simulink model "Model_LQR_Real_First_order"  (R2025a)
settings: Solver=ode4  StartTime=0.0  StopTime=2  FixedStep=0.0001  RelTol=1e-3
InitFcn:
  | addpath('functions');
model workspace: external: MATLAB File D:\OneDrive - University of Bristol\2025-2026\Major Project\LQR\LQR_First_order\Discrete_of_init_LQR.m (data not in the file)
values from neighbouring files (symbols this model uses):
  alpha_angle = 0.9    [Discrete_of_init_LQR.m]
  alpha_output = 0.71    [Discrete_of_init_LQR.m]
  c_omega = (N_gear^2 * Kt * Ke) / R_motor    (= 0.00492477886361)    [Discrete_of_init_LQR.m]    (also in init_LQR.m)
  c_V = (N_gear * Kt) / R_motor    (= 0.0277237642805)    [Discrete_of_init_LQR.m]    (also in init_LQR.m)
  dist_duration = 0    [L_curve.m]
  fric_1 = [f_v_1, f_c_1, k_fc_1]    [Discrete_of_init_LQR.m]    (also in furuta_single_inverted_pendulum_nonlive_copy.m; init_LQR.m)
  fric_arm = [f_v_arm, f_c_arm, k_fc_arm]    [Discrete_of_init_LQR.m]    (also in furuta_single_inverted_pendulum_nonlive_copy.m; init_LQR.m)
  I_1 = 1.1e-4    (= 0.00011)    [Discrete_of_init_LQR.m]    (also in furuta_single_A_B_matrices.m = in2(:,4); furuta_single_state_derivative.m = in4(:,4); init_LQR.m)
  I_arm = 7.39e-4    (= 0.000739)    [Discrete_of_init_LQR.m]    (also in furuta_single_A_B_matrices.m = in2(:,2); furuta_single_state_derivative.m = in4(:,2); init_LQR.m)
  init_S = [0; 0; 0.26; 0]    [Discrete_of_init_LQR.m]    (also in init_LQR.m)
  K_voltage = dlqr(G, H, Q, R)    [Discrete_of_init_LQR.m]    (also in init_LQR.m = lqr(A_new, B_new, Q, R))
  L_1 = 0.14    [Discrete_of_init_LQR.m]    (also in init_LQR.m; playback_animation_single.m = out.plotData.L_1.Data(1))
  L_arm = 0.1475    [Discrete_of_init_LQR.m]    (also in furuta_single_A_B_matrices.m = in2(:,1); furuta_single_state_derivative.m = in4(:,1); init_LQR.m; playback_animation_single.m = out.plotData.L_arm.Data(1))
  lcom_1 = 0.051    [Discrete_of_init_LQR.m]    (also in furuta_single_A_B_matrices.m = in2(:,3); furuta_single_state_derivative.m = in4(:,3); init_LQR.m; playback_animation_single.m = out.plotData.lcom_1.Data(1))
  m_1 = 0.054    [Discrete_of_init_LQR.m]    (also in furuta_single_A_B_matrices.m = in2(:,5); furuta_single_state_derivative.m = in4(:,5); init_LQR.m)
  t_dist = 999    [L_curve.m]    (also in stabilityanalysisplotting.m = 0.5)
libraries: simulink x4
settings Model: PacingRate=0.100000  Creator=Esther  LastModifiedBy=Hankin

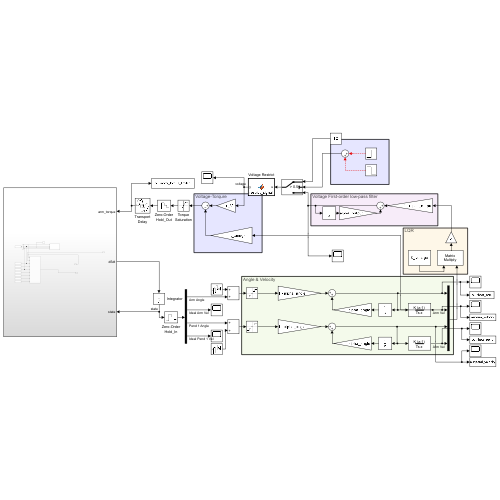
[thumbnail: Simulink's stored preview of the top-level diagram]
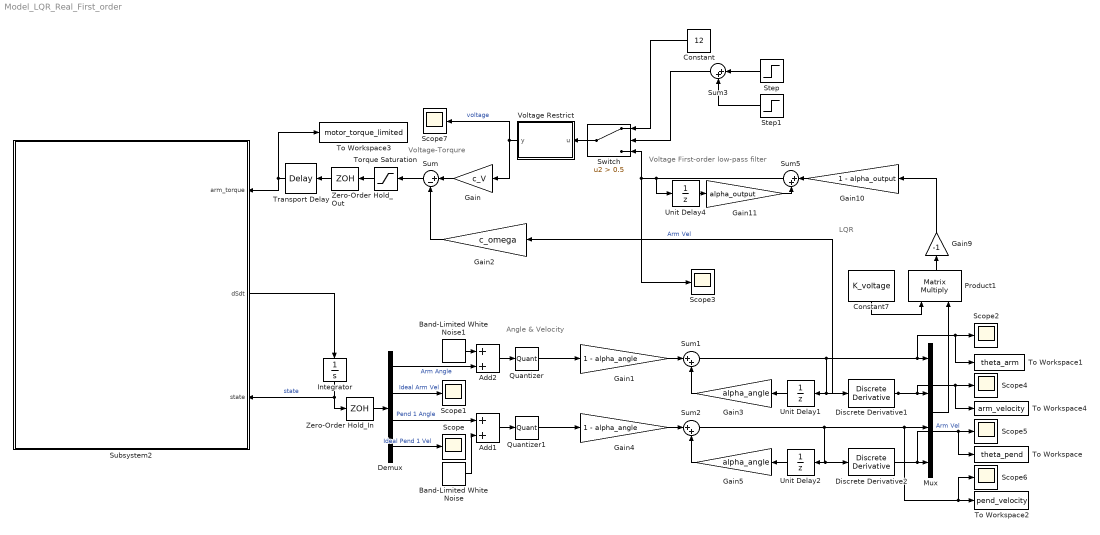
== system Model_LQR_Real_First_order ==
  note: Angle & Velocity
  note: Voltage-Torqure
  note: Voltage First-order low-pass filter
  note: LQR
  Add1 : Sum
  Add2 : Sum
  Band-Limited White Noise : simulink/Sources/Band-Limited White Noise  Cov=[1e-9]  Ts=0.001  seed=[23341]
  Band-Limited White Noise1 : simulink/Sources/Band-Limited White Noise  Cov=[1e-8]  Ts=0.001  seed=[23341]
  Constant : Constant  Value=12
  Constant7 : Constant  Value=K_voltage  VectorParams1D=off
  Demux : Demux
  Discrete Derivative1 : simulink/Discrete/Discrete Derivative  gainval=1.0  ICPrevScaledInput=0.0  OutMin=[]  OutMax=[]  OutDataType=fixdt(1, 16)  OutScaling=2^-10  DoSatur=off
  Discrete Derivative2 : simulink/Discrete/Discrete Derivative  gainval=1.0  ICPrevScaledInput=0.0  OutMin=[]  OutMax=[]  OutDataType=fixdt(1, 16)  OutScaling=2^-10  DoSatur=off
  Gain : Gain  Gain=c_V
  Gain1 : Gain  Gain=1 - alpha_angle
  Gain10 : Gain  Gain=1 - alpha_output
  Gain11 : Gain  Gain=alpha_output
  Gain2 : Gain  Gain=c_omega
  Gain3 : Gain  Gain=alpha_angle
  Gain4 : Gain  Gain=1 - alpha_angle
  Gain5 : Gain  Gain=alpha_angle
  Gain9 : Gain  Gain=-1
  Integrator : Integrator  InitialCondition=init_S
  Mux : Mux
  Product1 : Product  Multiplication=Matrix(*)
  Quantizer : Quantizer  QuantizationInterval=2*pi/408  LinearizeAsGain=off
  Quantizer1 : Quantizer  QuantizationInterval=2*pi/8000  LinearizeAsGain=off
  Scope{,1..7} (8 alike) : Scope
      Scope2 settings: ActiveDisplayYMinimum=-0.24013584318940978  ActiveDisplayYMaximum=0.31113568260293173  DataLoggingVariableName=ScopeData2
      Scope3 settings: ActiveDisplayYMinimum=-9.2448445777431179  ActiveDisplayYMaximum=10.619194990037117  DataLoggingVariableName=ScopeData3
      Scope4 settings: DataLoggingVariableName=ScopeData4
      Scope5 settings: ActiveDisplayYMinimum=-1  ActiveDisplayYMaximum=1  DataLoggingVariableName=ScopeData5
      Scope6 settings: ActiveDisplayYMinimum=-0.016550586353962036  ActiveDisplayYMaximum=0.035155299071454024  DataLoggingVariableName=ScopeData6
      Scope7 settings: ActiveDisplayYMinimum=-4.07418345548384  ActiveDisplayYMaximum=7.6194023262449049  DataLoggingVariableName=ScopeData7
  Step : Step  Time=t_dist  SampleTime=0  VectorParams1D=off
  Step1 : Step  Time=t_dist + dist_duration  After=-1  SampleTime=0  VectorParams1D=off
  Subsystem2 : Subsystem
      settings: PortSchema="{\"entries\":[{\"content\":{\"sides\":[{\"content\":{},\"type\":\"ConnectorPlacement.EquallySpacedRectSide\",\"uuid\":\"5bb040f9-7631-4ddd-98c9-47038337a419\"},{\"content\":{\"connectorIds\":[\"In1\",\"Out1\",\"In2\"],\"side\":\"RIGHT\"},\"type\":\"ConnectorPlacement.EquallySpacedRectSide\",\"uuid\":\"3aaaaaf2-68ad-4a58-822b-18678aa9886a\"},{\"content\":{\"side\":\"TOP\"},\"type\":\"ConnectorPlacement.EquallySpacedRectSide\",\"uuid\":\"9a08505c-87f2-40af-98ad-a65fb656621c\"}]},\"type\":\"ConnectorPlacement.EquallySpacedConnector\",\"uuid\":\"c01f2304-e45c-4dd4-b6eb-ff36d0bfa340\"}],\"packageUris\":[\"http://schema.mathworks.com/mf0/Connector/R2020b\"],\"version\":\"1.0\"}"
  Sum : Sum  Inputs=|+-
  Sum{1..3,5} (4 alike) : Sum  Inputs=|++
  Switch : Switch  Criteria=u2 > Threshold  Threshold=0.5  SaturateOnIntegerOverflow=off  InputSameDT=off
  To Workspace : ToWorkspace  VariableName=theta_pend  SaveFormat=Timeseries  SampleTime=-1
  To Workspace1 : ToWorkspace  VariableName=theta_arm  SaveFormat=Timeseries  SampleTime=-1
  To Workspace2 : ToWorkspace  VariableName=pend_velocity  SaveFormat=Timeseries  SampleTime=-1
  To Workspace3 : ToWorkspace  VariableName=motor_torque_limited  SaveFormat=Timeseries  SampleTime=-1
  To Workspace4 : ToWorkspace  VariableName=arm_velocity  SaveFormat=Timeseries  SampleTime=-1
  Torque Saturation : Saturate  UpperLimit=0.088  LowerLimit=-0.088  LinearizeAsGain=off
  Transport Delay : TransportDelay  DelayTime=0.01195
  Unit Delay1 : UnitDelay  InputProcessing=Columns as channels (frame based)  SampleTime=-1  HasFrameUpgradeWarning=on
  Unit Delay2 : UnitDelay  InputProcessing=Columns as channels (frame based)  SampleTime=-1  HasFrameUpgradeWarning=on
  Unit Delay4 : UnitDelay  InputProcessing=Columns as channels (frame based)  SampleTime=-1  HasFrameUpgradeWarning=on
  Voltage Restrict : MATLAB Function  TreatAsAtomicUnit=on
  Zero-Order Hold_In : ZeroOrderHold  SampleTime=0.001
  Zero-Order Hold_Out : ZeroOrderHold  SampleTime=0.001
  wires:
  Integrator/1 -> Zero-Order Hold_In/1, Subsystem2/2(state)  "state"
  Demux/1 -> Add2/2  "Arm Angle"
  Demux/3 -> Add1/1  "Pend 1 Angle"
  Zero-Order Hold_In/1 -> Demux/1
  Sum/1 -> Torque Saturation/1
  Zero-Order Hold_Out/1 -> Transport Delay/1
  Subsystem2/1(dSdt) -> Integrator/1
  Transport Delay/1 -> Subsystem2/1(arm_torque), To Workspace3/1
  Gain/1 -> Sum/1
  Gain2/1 -> Sum/2
  Band-Limited White Noise/1 -> Add1/2
  Add1/1 -> Quantizer1/1
  Add2/1 -> Quantizer/1
  Band-Limited White Noise1/1 -> Add2/1
  Demux/4 -> Scope/1  "Ideal Pend 1 Vel"
  Demux/2 -> Scope1/1  "Ideal Arm Vel"
  Constant7/1 -> Product1/1
  Unit Delay4/1 -> Gain11/1
  Gain10/1 -> Sum5/1
  Gain11/1 -> Sum5/2
  Product1/1 -> Gain9/1
  Voltage Restrict/1(y) -> Gain/1, Scope7/1  "voltage"
  Mux/1 -> Product1/2
  Torque Saturation/1 -> Zero-Order Hold_Out/1
  Discrete Derivative2/1 -> To Workspace/1, Scope5/1, Mux/4  "Arm Vel"
  Quantizer/1 -> Gain1/1
  Unit Delay1/1 -> Gain3/1
  Gain3/1 -> Sum1/2
  Gain1/1 -> Sum1/1
  Discrete Derivative1/1 -> To Workspace4/1, Scope4/1, Mux/2, Gain2/1  "Arm Vel"
  Gain5/1 -> Sum2/2
  Unit Delay2/1 -> Gain5/1
  Gain4/1 -> Sum2/1
  Quantizer1/1 -> Gain4/1
  Gain9/1 -> Gain10/1
  Sum1/1 -> Unit Delay1/1, Discrete Derivative1/1, Scope2/1, To Workspace1/1, Mux/1
  Sum2/1 -> Unit Delay2/1, Discrete Derivative2/1, Scope6/1, To Workspace2/1, Mux/3
  Step/1 -> Sum3/1
  Step1/1 -> Sum3/2
  Sum5/1 -> Unit Delay4/1, Switch/3, Scope3/1
  Switch/1 -> Voltage Restrict/1(u)
  Sum3/1 -> Switch/2
  Constant/1 -> Switch/1

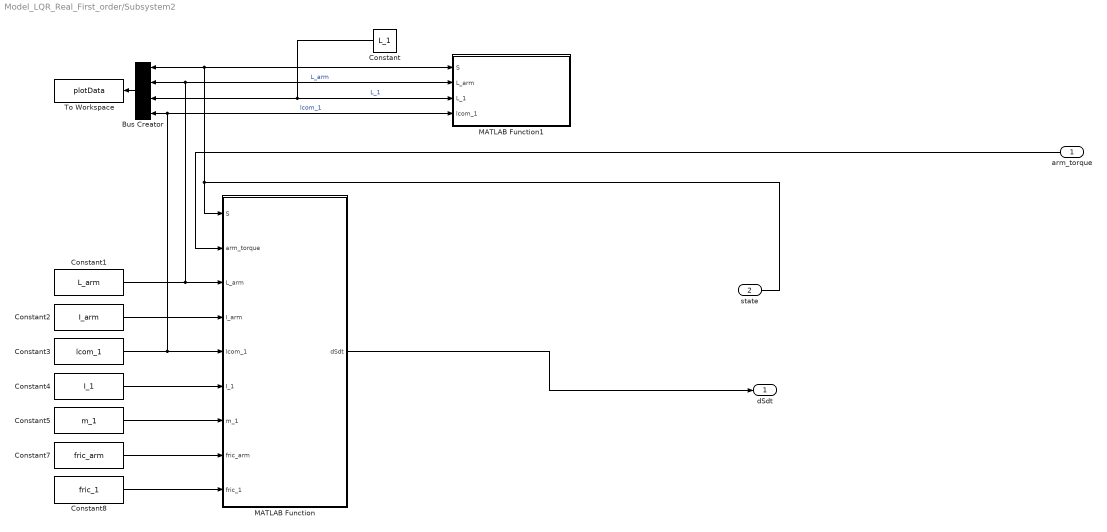
== system Model_LQR_Real_First_order/Subsystem2 ==
  arm_torque : Inport
  state : Inport  Port=2
  Bus Creator : BusCreator  Inputs=4
  Constant : Constant  Value=L_1
  Constant1 : Constant  Value=L_arm
  Constant2 : Constant  Value=I_arm
  Constant3 : Constant  Value=lcom_1
  Constant4 : Constant  Value=I_1
  Constant5 : Constant  Value=m_1
  Constant7 : Constant  Value=fric_arm  VectorParams1D=off
  Constant8 : Constant  Value=fric_1  VectorParams1D=off
  MATLAB Function : MATLAB Function  TreatAsAtomicUnit=on
  MATLAB Function1 : MATLAB Function  TreatAsAtomicUnit=on
  To Workspace : ToWorkspace  VariableName=plotData  SaveFormat=Timeseries  SampleTime=-1
  dSdt : Outport
  wires:
  Constant3/1 -> Bus Creator/4, MATLAB Function1/4(lcom_1), MATLAB Function/5(lcom_1)  "lcom_1"
  Constant1/1 -> Bus Creator/2, MATLAB Function1/2(L_arm), MATLAB Function/3(L_arm)  "L_arm"
  Constant7/1 -> MATLAB Function/8(fric_arm)
  MATLAB Function/1(dSdt) -> dSdt/1
  Constant/1 -> MATLAB Function1/3(L_1), Bus Creator/3  "L_1"
  Constant2/1 -> MATLAB Function/4(I_arm)
  Constant8/1 -> MATLAB Function/9(fric_1)
  state/1 -> Bus Creator/1, MATLAB Function1/1(S), MATLAB Function/1(S)
  Constant5/1 -> MATLAB Function/7(m_1)
  Bus Creator/1 -> To Workspace/1
  Constant4/1 -> MATLAB Function/6(I_1)
  arm_torque/1 -> MATLAB Function/2(arm_torque)

== matlab function Model_LQR_Real_First_order/Subsystem2/MATLAB Function1 ==
  settings: updateMethod=DISCRETE
  data: S input; L_arm input; L_1 input; lcom_1 input
function animation(S, L_arm, L_1, lcom_1)
    update_ratio = 100;
    realtime_animation_single(S, L_arm, L_1, lcom_1, update_ratio);
end

== matlab function Model_LQR_Real_First_order/Subsystem2/MATLAB Function ==
  data: S input size=4; dSdt output size=4; arm_torque input size=1; L_arm input size=1; I_arm input size=1; lcom_1 input size=1; I_1 input size=1; m_1 input size=1; fric_arm input; fric_1 input
function dSdt = get_dSdt(S, arm_torque, L_arm, I_arm, lcom_1, I_1, m_1, fric_arm, fric_1)
    t = 0;
    g = 9.81;
    phys_param = [L_arm, I_arm, lcom_1, I_1, m_1, g];
    dSdt = furuta_single_state_derivative(t, S, arm_torque, phys_param, fric_arm, fric_1);
end

== matlab function Model_LQR_Real_First_order/Voltage Restrict ==
  data: u input; y output
function y = restrict_signal(u)
      % 限制最大值和最小值
      if u > 12
          y = 12;
      elseif u < -12
          y = -12;
      % 限制中心剔除区间 (-0.6, 0.6)
      % 将非负微小信号钳位至正区间下限
      elseif u >= 0 && u < 0.6
          y = 0;
      % 将负微小信号钳位至负区间上限
      elseif u < 0 && u > -0.6
          y = 0;
      % 信号在正常区间 [-12, -0.6] 或 [0.6, 12] 内，保持原值
      else
          y = u;
      end
  end
